simulink model "aeropendulo_pid"  (R2026a)
settings: Solver=ode45  StopTime=sum(p.sec_dur) - p.Ts  MaxStep=1e-3
PreLoadFcn:
  | p = parametros();
libraries: slpidlib x1, simulink x1
settings Model: Creator=sebastian  LastModifiedBy=sebastian

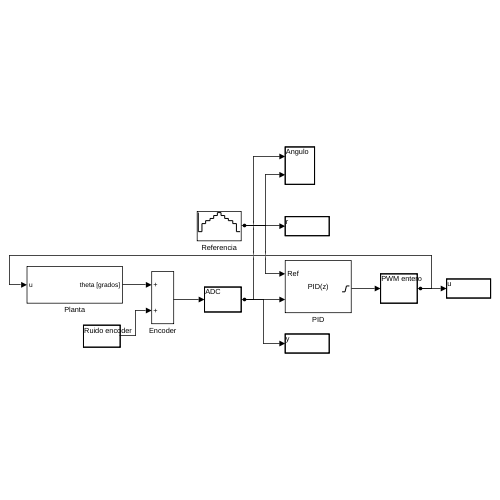
[thumbnail: Simulink's stored preview of the top-level diagram]
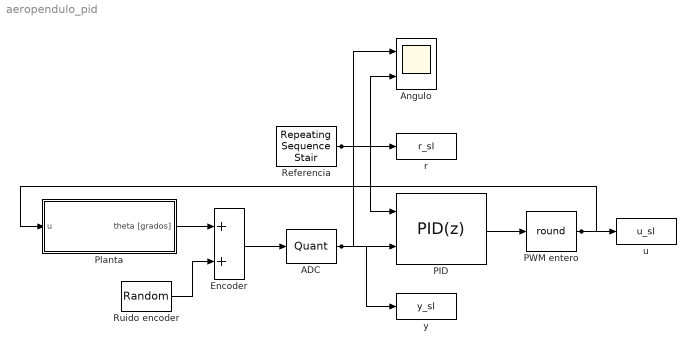
== system aeropendulo_pid ==
  ADC : Quantizer  QuantizationInterval=p.q_theta
  Angulo : Scope  NumInputPorts=2
  Encoder : Sum
  PID : slpidlib/PID Controller (2DOF)  Controller=PID  Form=Parallel  TimeDomain=Discrete-time  UseExternalTs=off  SampleTime=p.Ts  IntegratorMethod=Trapezoidal  FilterMethod=Trapezoidal  ControllerParametersSource=internal  P=p.Kp  I=p.Ki  UseKiTs=off  D=p.Kd  UseExternalDerivativeSource=off  N=1/p.Tf  UseFilter=on  b=p.beta  c=0  TunerSelectOption=Transfer Function Based (PID Tuner App)  InitialConditionSource=internal  InitialConditionForIntegrator=0  InitialConditionForFilter=0  DifferentiatorICPrevScaledInput=0  ExternalReset=none  TrackingMode=off  Kt=1  LimitOutput=on  SatLimitsSource=internal  UpperSaturationLimit=p.u_max  LowerSaturationLimit=0  LinearizeAsGain=on  AntiWindupMode=clamping  Kb=1  LimitIntegrator=off  UpperIntegratorSaturationLimit=inf  LowerIntegratorSaturationLimit=-inf  POutMin=[]  POutMax=[]  IOutMin=[]  IOutMax=[]  DOutMin=[]  DOutMax=[]  NOutMin=[]  NOutMax=[]  bOutMin=[]  bOutMax=[]  cOutMin=[]  cOutMax=[]  SumOutMin=[]  SumOutMax=[]  SaturationOutMin=[]  SaturationOutMax=[]  PParamMin=[]  PParamMax=[]  IParamMin=[]  IParamMax=[]  DParamMin=[]  DParamMax=[]  NParamMin=[]  NParamMax=[]  bParamMin=[]  bParamMax=[]  cParamMin=[]  cParamMax=[]  KbParamMin=[]  KbParamMax=[]  KtParamMin=[]  KtParamMax=[]  KbOutMin=[]  KbOutMax=[]  KtOutMin=[]  KtOutMax=[]  IntegratorOutMin=[]  IntegratorOutMax=[]  FilterOutMin=[]  FilterOutMax=[]  SumI1OutMin=[]  SumI1OutMax=[]  SumI2OutMin=[]  SumI2OutMax=[]  SumI3OutMin=[]  SumI3OutMax=[]  SumI4OutMin=[]  SumI4OutMax=[]  SumDOutMin=[]  SumDOutMax=[]  Sum1OutMin=[]  Sum1OutMax=[]  Sum2OutMin=[]  Sum2OutMax=[]  Sum3OutMin=[]  Sum3OutMax=[]  DifferentiatorOutMin=[]  DifferentiatorOutMax=[]  FilterDiffOutCoefMin=[]  FilterDiffOutCoefMax=[]  ReciprocalOutMin=[]  ReciprocalOutMax=[]  SumDenOutMin=[]  SumDenOutMax=[]  SumNumOutMin=[]  SumNumOutMax=[]  DivideOutMin=[]  DivideOutMax=[]  UdiffTsProdOutMin=[]  UdiffTsProdOutMax=[]  NTsProdOutMin=[]  NTsProdOutMax=[]  UintegralTsProdOutMin=[]  UintegralTsProdOutMax=[]  UngainTsProdOutMin=[]  UngainTsProdOutMax=[]  ClampingZeroOutDataTypeStr=Inherit: Inherit via back propagation  ClampingZeroOutMin=[]  ClampingZeroOutMax=[]  FilterDenConstantOutDataTypeStr=Inherit: Inherit via back propagation  FilterDenConstantOutMin=[]  FilterDenConstantOutMax=[]  PCopyOutDataTypeStr=Inherit: Inherit via back propagation  PCopyOutMin=[]  PCopyOutMax=[]  NCopyOutDataTypeStr=Inherit: Inherit via back propagation  NCopyOutMin=[]  NCopyOutMax=[]  IntegratorContinuousStateAttributes=''  IntegratorStateMustResolveToSignalObject=off  IntegratorRTWStateStorageClass=Auto  FilterContinuousStateAttributes=''  FilterStateMustResolveToSignalObject=off  FilterRTWStateStorageClass=Auto  ParallelPVariant=InternalParameters  IdealPVariant=Disabled  IVariant=InternalParameters  DVariant=InternalParameters  bVariant=InternalParameters  cVariant=InternalParameters  IntegratorVariant=Discrete  SatVariant=Enabled  AWVariant=DiscClampingParallel  PCopyVariant=Disabled  TRVariant=Disabled  FdbkBlocksVariant=Feedback  IdealPFdbkVariant=Passthrough  SatFdbkVariant=Passthrough  DerivativeFilterVariant=TrapezoidalFilter  NVariant=InternalParameters  NCopyVariant=InternalParameters  FilterICVariant=InternalICsFilter  IntegratorICVariant=InternalICs  ExternalResetVariant=Disabled  TRSumVariant=Passthrough  SumFdbkVariant=Enabled  SumVariant=Sum_PID  TsampFilterVariant=InternalTs  TsampNgainVariant=Passthrough  TsampIntegralVariant=Disabled_SignalSpec  ExternalSaturationOutDataTypeStr=Inherit: Same as second input  DerivativeSourceVariant=ErrorSignal  PreIntVariant=InternalPreInt
  PWM entero : Rounding  Operator=round
  Planta : Subsystem
  Referencia : simulink/Sources/Repeating Sequence Stair  OutValues=p.sec_ref  tsamp=p.sec_dur(1)  OutMin=[]  OutMax=[]  OutDataTypeStr=double  OutputDataTypeScalingMode=double  OutDataType=fixdt(0,8)  ConRadixGroup=Best Precision: Vector-wise  OutScaling=2^-12
  Ruido encoder : RandomNumber  Variance=p.sigma_theta^2  Seed=1  SampleTime=p.Ts
  r : ToWorkspace  VariableName=r_sl  SaveFormat=Timeseries  SampleTime=-1
  u : ToWorkspace  VariableName=u_sl  SaveFormat=Timeseries  SampleTime=-1
  y : ToWorkspace  VariableName=y_sl  SaveFormat=Timeseries  SampleTime=-1
  wires:
  PWM entero/1 -> u/1, Planta/1(u)
  PID/1 -> PWM entero/1
  ADC/1 -> Angulo/1, y/1, PID/2
  Referencia/1 -> Angulo/2, r/1, PID/1
  Encoder/1 -> ADC/1
  Ruido encoder/1 -> Encoder/2
  Planta/1(theta [grados]) -> Encoder/1

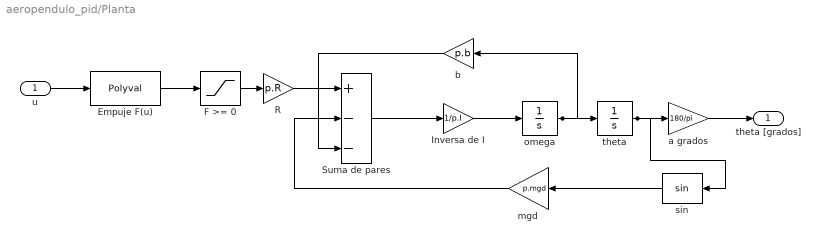
== system aeropendulo_pid/Planta ==
  u : Inport
  Empuje F(u) : Polyval  Coefs=p.Fcuad
  F >= 0 : Saturate  UpperLimit=inf  LowerLimit=0
  Inversa de I : Gain  Gain=1/p.I
  R : Gain  Gain=p.R
  Suma de pares : Sum  Inputs=+--
  a grados : Gain  Gain=180/pi
  b : Gain  Gain=p.b
  mgd : Gain  Gain=p.mgd
  omega : Integrator
  sin : Trigonometry
  theta : Integrator
  theta [grados] : Outport
  wires:
  theta/1 -> a grados/1, sin/1
  omega/1 -> theta/1, b/1
  mgd/1 -> Suma de pares/2
  Inversa de I/1 -> omega/1
  sin/1 -> mgd/1
  b/1 -> Suma de pares/3
  Suma de pares/1 -> Inversa de I/1
  R/1 -> Suma de pares/1
  F >= 0/1 -> R/1
  Empuje F(u)/1 -> F >= 0/1
  a grados/1 -> theta [grados]/1
  u/1 -> Empuje F(u)/1
